simulink model "Balancing_Robot_Nominal"  (R2024b)
settings: Solver=VariableStepAuto  StartTime=0.0  StopTime=10.0  RelTol=1e-3
undefined symbols (not defined in the file): C_filter, drv, dspblkCoreblockFVToolHelper, gbox, gcbh, K_Nom_LQR_Br, Nu, Nx, sens, T, wheel
settings Model: Creator=liliy  LastModifiedBy=liliy

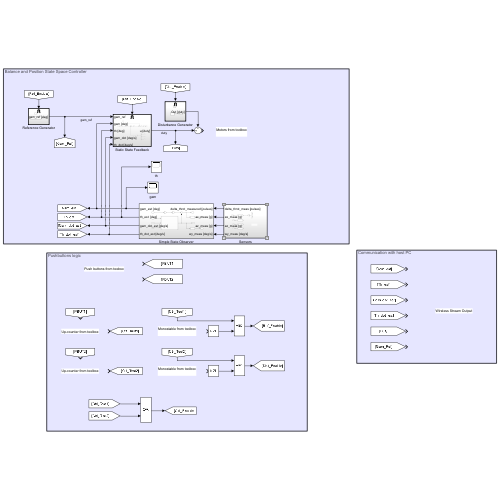
[thumbnail: Simulink's stored preview of the top-level diagram]
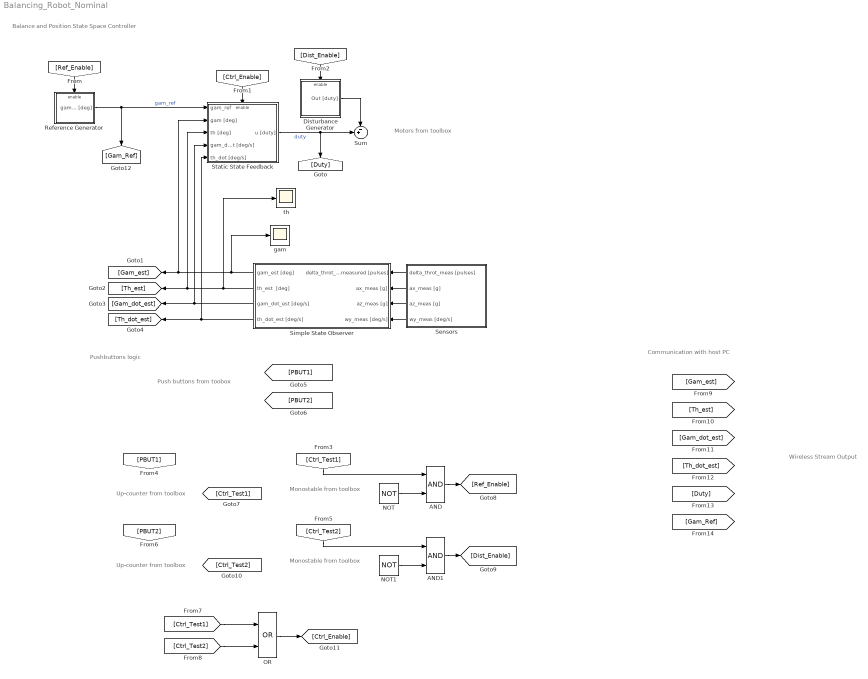
== system Balancing_Robot_Nominal ==
  note: Balance and Position State Space Controller
  note: Communication with host PC
  note: Wireless Stream Output
  note: Pushbuttons logic
  note: Monostable from toolbox
  note: Up-counter from toolbox
  note: Push buttons from toobox
  note: Motors from toolbox
  note: Monostable from toolbox
  note: Up-counter from toolbox
  AND : Logic  AllPortsSameDT=off  OutDataTypeStr=boolean
  AND1 : Logic  AllPortsSameDT=off  OutDataTypeStr=boolean
  Disturbance Generator : Subsystem
  NOT : Logic  Operator=NOT  AllPortsSameDT=off  OutDataTypeStr=boolean
  NOT1 : Logic  Operator=NOT  AllPortsSameDT=off  OutDataTypeStr=boolean
  OR : Logic  Operator=OR  AllPortsSameDT=off  OutDataTypeStr=boolean
  Reference Generator : Subsystem
  Sensors : Subsystem
  Simple State Observer : Subsystem
  Static State Feedback : Subsystem
  Sum : Sum  Inputs=-+|
  gam : Scope
  th : Scope
  wires:
  Static State Feedback/1(u [duty]) -> Sum/2, [Duty]  "duty"
  Reference Generator/1(gam_ref [deg]) -> [Gam_Ref], Static State Feedback/1(gam_ref)  "gam_ref"
  Simple State Observer/4(th_dot_est [deg/s]) -> Static State Feedback/5(th_dot [deg/s]), [Th_dot_est]
  Simple State Observer/3(gam_dot_est [deg/s]) -> Static State Feedback/4(gam_dot [deg/s]), [Gam_dot_est]
  Simple State Observer/2(th_est  [deg]) -> th/1, Static State Feedback/3(th [deg]), [Th_est]
  Simple State Observer/1(gam_est [deg]) -> gam/1, Static State Feedback/2(gam [deg]), [Gam_est]
  [Ref_Enable] -> Reference Generator/Enable
  [Ctrl_Enable] -> Static State Feedback/Enable
  Disturbance Generator/1(Out [duty]) -> Sum/1
  [Dist_Enable] -> Disturbance Generator/Enable
  Sensors/4(wy_meas [deg/s]) -> Simple State Observer/4(wy_meas [deg/s])
  Sensors/3(az_meas [g]) -> Simple State Observer/3(az_meas [g])
  Sensors/2(ax_meas [g]) -> Simple State Observer/2(ax_meas [g])
  Sensors/1(delta_throt_meas [pulses]) -> Simple State Observer/1(delta_throt_measured [pulses])
  [Ctrl_Test1] -> AND/1
  NOT/1 -> AND/2
  AND/1 -> [Ref_Enable]
  AND1/1 -> [Dist_Enable]
  NOT1/1 -> AND1/2
  [Ctrl_Test2] -> AND1/1
  [Ctrl_Test2] -> OR/2
  [Ctrl_Test1] -> OR/1
  OR/1 -> [Ctrl_Enable]

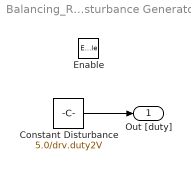
== system Balancing_Robot_Nominal/Disturbance Generator ==
  Enable : EnablePort
  Constant Disturbance : Constant  Value=5.0/drv.duty2V
  Out [duty] : Outport
  wires:
  Constant Disturbance/1 -> Out [duty]/1

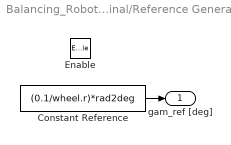
== system Balancing_Robot_Nominal/Reference Generator ==
  Enable : EnablePort
  Constant Reference : Constant  Value=(0.1/wheel.r)*rad2deg
  gam_ref [deg] : Outport
  wires:
  Constant Reference/1 -> gam_ref [deg]/1

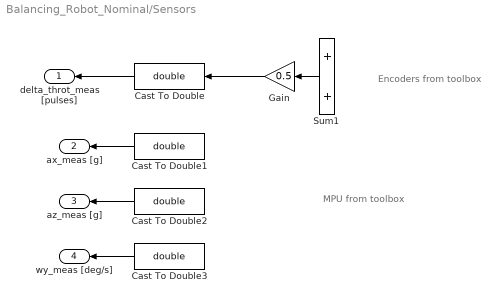
== system Balancing_Robot_Nominal/Sensors ==
  note: Encoders from toolbox
  note: MPU from toolbox
  Cast To Double{,1..3} (4 alike) : DataTypeConversion  OutDataTypeStr=double  SaturateOnIntegerOverflow=off  RndMeth=Floor
  Gain : Gain  Gain=0.5
  Sum1 : Sum
  delta_throt_meas [pulses] : Outport
  ax_meas [g] : Outport  Port=2
  az_meas [g] : Outport  Port=3
  wy_meas [deg/s] : Outport  Port=4
  wires:
  Sum1/1 -> Gain/1
  Gain/1 -> Cast To Double/1
  Cast To Double/1 -> delta_throt_meas [pulses]/1
  Cast To Double3/1 -> wy_meas [deg/s]/1
  Cast To Double2/1 -> az_meas [g]/1
  Cast To Double1/1 -> ax_meas [g]/1

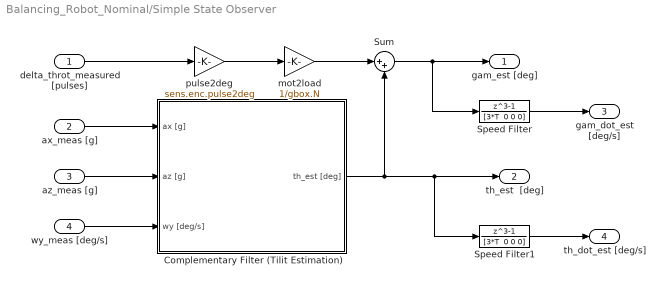
== system Balancing_Robot_Nominal/Simple State Observer ==
  delta_throt_measured [pulses] : Inport
  ax_meas [g] : Inport  Port=2
  az_meas [g] : Inport  Port=3
  wy_meas [deg/s] : Inport  Port=4
  Complementary Filter (Tilit Estimation) : Subsystem
  Speed Filter : DiscreteTransferFcn  LoadFcn=dspblkCoreblockFVToolHelper(gcbh,'load');  Numerator=[1 0 0 -1]  Denominator="[3*T  0 0 0]"
      settings: CopyFcn=dspblkCoreblockFVToolHelper(gcbh,'copy');  DeleteFcn=dspblkCoreblockFVToolHelper(gcbh,'close');  ModelCloseFcn=dspblkCoreblockFVToolHelper(gcbh,'close');  PreSaveFcn=dspblkCoreblockFVToolHelper(gcbh,'presave');  PostSaveFcn=dspblkCoreblockFVToolHelper(gcbh,'postsave');  CloseFcn=dspblkCoreblockFVToolHelper(gcbh,'close');
  Speed Filter1 : DiscreteTransferFcn  LoadFcn=dspblkCoreblockFVToolHelper(gcbh,'load');  Numerator=[1 0 0 -1]  Denominator="[3*T  0 0 0]"
      settings: CopyFcn=dspblkCoreblockFVToolHelper(gcbh,'copy');  DeleteFcn=dspblkCoreblockFVToolHelper(gcbh,'close');  ModelCloseFcn=dspblkCoreblockFVToolHelper(gcbh,'close');  PreSaveFcn=dspblkCoreblockFVToolHelper(gcbh,'presave');  PostSaveFcn=dspblkCoreblockFVToolHelper(gcbh,'postsave');  CloseFcn=dspblkCoreblockFVToolHelper(gcbh,'close');
  Sum : Sum  Inputs=|++
  mot2load : Gain  Gain=1/gbox.N
  pulse2deg : Gain  Gain=sens.enc.pulse2deg
  gam_est [deg] : Outport
  th_est  [deg] : Outport  Port=2
  gam_dot_est [deg/s] : Outport  Port=3
  th_dot_est [deg/s] : Outport  Port=4
  wires:
  mot2load/1 -> Sum/1
  Complementary Filter (Tilit Estimation)/1(th_est [deg]) -> th_est  [deg]/1, Speed Filter1/1, Sum/2
  Speed Filter1/1 -> th_dot_est [deg/s]/1
  delta_throt_measured [pulses]/1 -> pulse2deg/1
  Speed Filter/1 -> gam_dot_est [deg/s]/1
  pulse2deg/1 -> mot2load/1
  Sum/1 -> gam_est [deg]/1, Speed Filter/1
  ax_meas [g]/1 -> Complementary Filter (Tilit Estimation)/1(ax [g])
  az_meas [g]/1 -> Complementary Filter (Tilit Estimation)/2(az [g])
  wy_meas [deg/s]/1 -> Complementary Filter (Tilit Estimation)/3(wy [deg/s])

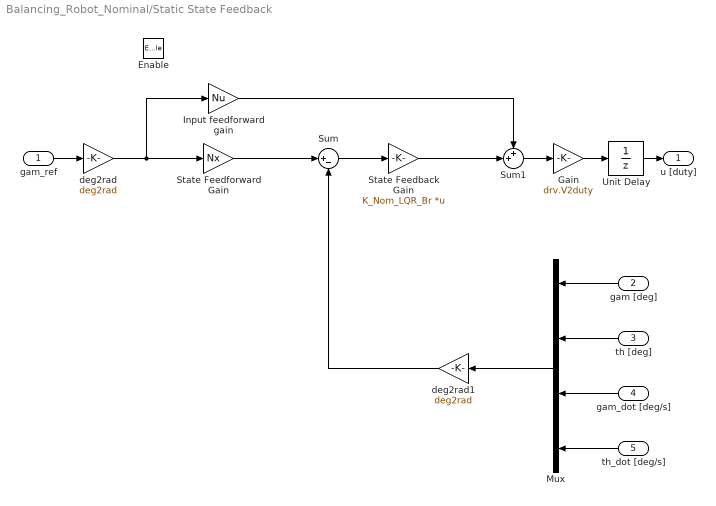
== system Balancing_Robot_Nominal/Static State Feedback ==
  gam_ref : Inport
  gam [deg] : Inport  Port=2
  th [deg] : Inport  Port=3
  gam_dot [deg/s] : Inport  Port=4
  th_dot [deg/s] : Inport  Port=5
  Enable : EnablePort
  Gain : Gain  Gain=drv.V2duty
  Input feedforward gain : Gain  Gain=Nu
  Mux : Mux
  State Feedback Gain : Gain  Gain=K_Nom_LQR_Br  Multiplication=Matrix(K*u)
  State Feedforward Gain : Gain  Gain=Nx
  Sum : Sum  Inputs=|+-
  Sum1 : Sum  Inputs=++|
  Unit Delay : UnitDelay  SampleTime=T  HasFrameUpgradeWarning=on
  deg2rad : Gain  Gain=deg2rad
  deg2rad1 : Gain  Gain=deg2rad
  u [duty] : Outport
  wires:
  Unit Delay/1 -> u [duty]/1
  deg2rad1/1 -> Sum/2
  th [deg]/1 -> Mux/2
  gam [deg]/1 -> Mux/1
  Gain/1 -> Unit Delay/1
  th_dot [deg/s]/1 -> Mux/4
  gam_dot [deg/s]/1 -> Mux/3
  Mux/1 -> deg2rad1/1
  Sum1/1 -> Gain/1
  Input feedforward gain/1 -> Sum1/1
  State Feedback Gain/1 -> Sum1/2
  Sum/1 -> State Feedback Gain/1
  State Feedforward Gain/1 -> Sum/1
  deg2rad/1 -> State Feedforward Gain/1, Input feedforward gain/1
  gam_ref/1 -> deg2rad/1

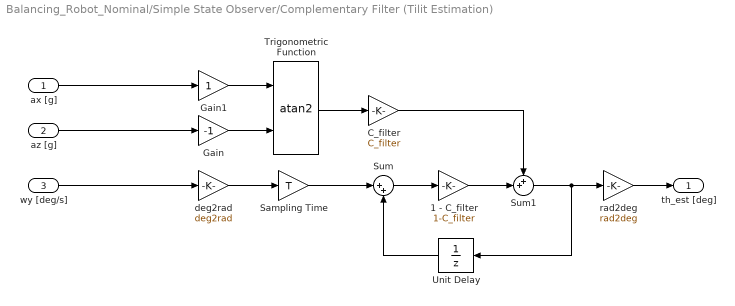
== system Balancing_Robot_Nominal/Simple State Observer/Complementary Filter (Tilit Estimation) ==
  ax [g] : Inport
  az [g] : Inport  Port=2
  wy [deg/s] : Inport  Port=3
  1 - C_filter : Gain  Gain=1-C_filter
  C_filter : Gain  Gain=C_filter
  Gain : Gain  Gain=-1
  Gain1 : Gain
  Sampling Time : Gain  Gain=T
  Sum : Sum  Inputs=|++
  Sum1 : Sum  Inputs=++|
  Trigonometric Function : Trigonometry  Operator=atan2
  Unit Delay : UnitDelay  SampleTime=T  HasFrameUpgradeWarning=on
  deg2rad : Gain  Gain=deg2rad
  rad2deg : Gain  Gain=rad2deg
  th_est [deg] : Outport
  wires:
  Trigonometric Function/1 -> C_filter/1
  Gain/1 -> Trigonometric Function/2
  rad2deg/1 -> th_est [deg]/1
  deg2rad/1 -> Sampling Time/1
  Sum/1 -> 1 - C_filter/1
  Gain1/1 -> Trigonometric Function/1
  Sum1/1 -> Unit Delay/1, rad2deg/1
  Sampling Time/1 -> Sum/1
  1 - C_filter/1 -> Sum1/2
  Unit Delay/1 -> Sum/2
  C_filter/1 -> Sum1/1
  ax [g]/1 -> Gain1/1
  az [g]/1 -> Gain/1
  wy [deg/s]/1 -> deg2rad/1
